simulink model "CoolingPredictiveMaintenance"  (R2024a)
settings: Solver=VariableStepAuto  StartTime=0.0  StopTime=10.0  RelTol=1e-3
settings Model: Creator=deshm  LastModifiedBy=deshm

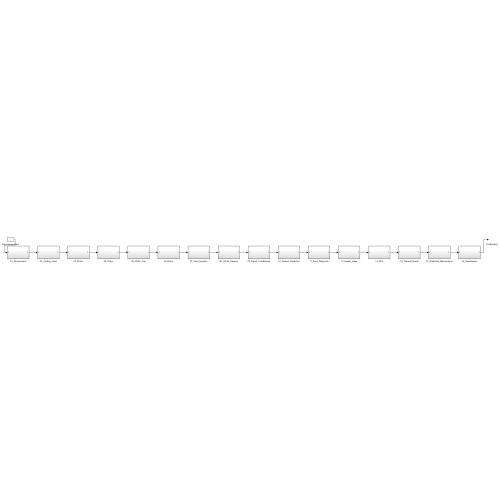
[thumbnail: Simulink's stored preview of the top-level diagram]
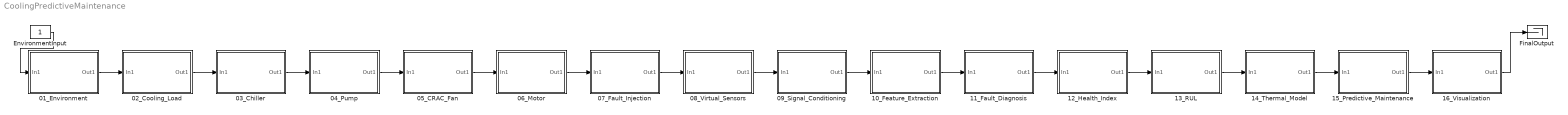
== system CoolingPredictiveMaintenance ==
  01_Environment : Subsystem
  02_Cooling_Load : Subsystem
  03_Chiller : Subsystem
  04_Pump : Subsystem
  05_CRAC_Fan : Subsystem
  06_Motor : Subsystem
  07_Fault_Injection : Subsystem
  08_Virtual_Sensors : Subsystem
  09_Signal_Conditioning : Subsystem
  10_Feature_Extraction : Subsystem
  11_Fault_Diagnosis : Subsystem
  12_Health_Index : Subsystem
  13_RUL : Subsystem
  14_Thermal_Model : Subsystem
  15_Predictive_Maintenance : Subsystem
  16_Visualization : Subsystem
  EnvironmentInput : Constant
  FinalOutput : Terminator
  wires:
  01_Environment/1(Out1) -> 02_Cooling_Load/1(In1)
  02_Cooling_Load/1(Out1) -> 03_Chiller/1(In1)
  03_Chiller/1(Out1) -> 04_Pump/1(In1)
  04_Pump/1(Out1) -> 05_CRAC_Fan/1(In1)
  05_CRAC_Fan/1(Out1) -> 06_Motor/1(In1)
  06_Motor/1(Out1) -> 07_Fault_Injection/1(In1)
  07_Fault_Injection/1(Out1) -> 08_Virtual_Sensors/1(In1)
  08_Virtual_Sensors/1(Out1) -> 09_Signal_Conditioning/1(In1)
  09_Signal_Conditioning/1(Out1) -> 10_Feature_Extraction/1(In1)
  10_Feature_Extraction/1(Out1) -> 11_Fault_Diagnosis/1(In1)
  11_Fault_Diagnosis/1(Out1) -> 12_Health_Index/1(In1)
  12_Health_Index/1(Out1) -> 13_RUL/1(In1)
  13_RUL/1(Out1) -> 14_Thermal_Model/1(In1)
  14_Thermal_Model/1(Out1) -> 15_Predictive_Maintenance/1(In1)
  15_Predictive_Maintenance/1(Out1) -> 16_Visualization/1(In1)
  EnvironmentInput/1 -> 01_Environment/1(In1)
  16_Visualization/1(Out1) -> FinalOutput/1

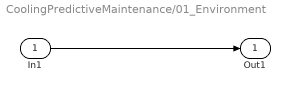
== system CoolingPredictiveMaintenance/01_Environment ==
  In1 : Inport
  Out1 : Outport
  wires:
  In1/1 -> Out1/1

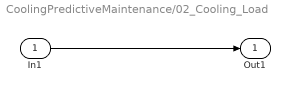
== system CoolingPredictiveMaintenance/02_Cooling_Load ==
  In1 : Inport
  Out1 : Outport
  wires:
  In1/1 -> Out1/1

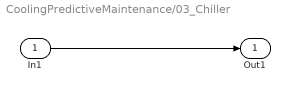
== system CoolingPredictiveMaintenance/03_Chiller ==
  In1 : Inport
  Out1 : Outport
  wires:
  In1/1 -> Out1/1

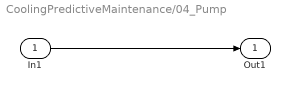
== system CoolingPredictiveMaintenance/04_Pump ==
  In1 : Inport
  Out1 : Outport
  wires:
  In1/1 -> Out1/1

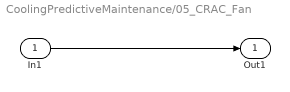
== system CoolingPredictiveMaintenance/05_CRAC_Fan ==
  In1 : Inport
  Out1 : Outport
  wires:
  In1/1 -> Out1/1

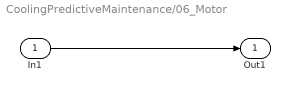
== system CoolingPredictiveMaintenance/06_Motor ==
  In1 : Inport
  Out1 : Outport
  wires:
  In1/1 -> Out1/1

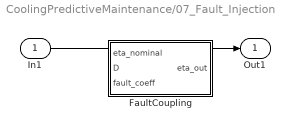
== system CoolingPredictiveMaintenance/07_Fault_Injection ==
  In1 : Inport
  FaultCoupling : MATLAB Function  TreatAsAtomicUnit=on
  Out1 : Outport
  wires:
  In1/1 -> Out1/1

== system CoolingPredictiveMaintenance/08_Virtual_Sensors ==
  In1 : Inport
  Out1 : Outport
  wires:
  In1/1 -> Out1/1

== system CoolingPredictiveMaintenance/09_Signal_Conditioning ==
  In1 : Inport
  Out1 : Outport
  wires:
  In1/1 -> Out1/1

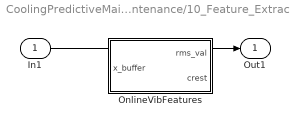
== system CoolingPredictiveMaintenance/10_Feature_Extraction ==
  In1 : Inport
  OnlineVibFeatures : MATLAB Function  TreatAsAtomicUnit=on
  Out1 : Outport
  wires:
  In1/1 -> Out1/1

== system CoolingPredictiveMaintenance/11_Fault_Diagnosis ==
  In1 : Inport
  Out1 : Outport
  wires:
  In1/1 -> Out1/1

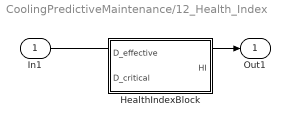
== system CoolingPredictiveMaintenance/12_Health_Index ==
  In1 : Inport
  HealthIndexBlock : MATLAB Function  TreatAsAtomicUnit=on
  Out1 : Outport
  wires:
  In1/1 -> Out1/1

== system CoolingPredictiveMaintenance/13_RUL ==
  In1 : Inport
  Out1 : Outport
  wires:
  In1/1 -> Out1/1

== system CoolingPredictiveMaintenance/14_Thermal_Model ==
  In1 : Inport
  Out1 : Outport
  wires:
  In1/1 -> Out1/1

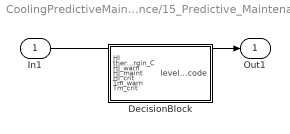
== system CoolingPredictiveMaintenance/15_Predictive_Maintenance ==
  In1 : Inport
  DecisionBlock : MATLAB Function  TreatAsAtomicUnit=on
  Out1 : Outport
  wires:
  In1/1 -> Out1/1

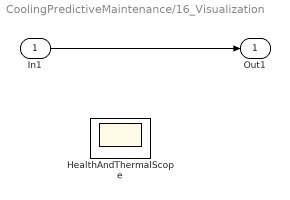
== system CoolingPredictiveMaintenance/16_Visualization ==
  In1 : Inport
  HealthAndThermalScope : Scope
  Out1 : Outport
  wires:
  In1/1 -> Out1/1

== matlab function CoolingPredictiveMaintenance/10_Feature_Extraction/OnlineVibFeatures ==
  data: x_buffer input; rms_val output; crest output
function [rms_val, crest] = OnlineVibFeatures(x_buffer)
%#codegen
% Simulink-native subset of src/features/extract_vibration_features.m
% (time-domain only, for real-time use inside the model).
rms_val = sqrt(mean(x_buffer.^2));
peak = max(abs(x_buffer));
crest = peak / max(rms_val, eps);
end

== matlab function CoolingPredictiveMaintenance/07_Fault_Injection/FaultCoupling ==
  data: eta_nominal input; eta_out output; D input; fault_coeff input
function eta_out = FaultCoupling(eta_nominal, D, fault_coeff)
%#codegen
% Re-expresses the generic degradation coupling from
% src/faults/apply_pump_fault.m / apply_fan_fault.m:
%   eta_fault = eta_nominal * (1 - fault_coeff*D)
eta_out = eta_nominal * (1 - fault_coeff*D);
end

== matlab function CoolingPredictiveMaintenance/12_Health_Index/HealthIndexBlock ==
  data: D_effective input; HI output; D_critical input
function HI = HealthIndexBlock(D_effective, D_critical)
%#codegen
% Re-expresses src/health_index/compute_health_index.m
norm_score = min(max(D_effective / D_critical, 0), 1);
HI = 100 * (1 - norm_score);
end

== matlab function CoolingPredictiveMaintenance/15_Predictive_Maintenance/DecisionBlock ==
  data: HI input; level_code output; thermal_margin_C input; HI_warn input; HI_maint input; HI_crit input; Tm_warn input; Tm_crit input
function level_code = DecisionBlock(HI, thermal_margin_C, HI_warn, HI_maint, HI_crit, Tm_warn, Tm_crit)
%#codegen
% Re-expresses the escalation logic in
% src/maintenance/maintenance_decision_engine.m as a numeric code:
% 0=NORMAL 1=MONITOR 2=WARNING 3=MAINTENANCE_REQUIRED 4=CRITICAL
level_code = 0;
if HI <= HI_crit
    level_code = 4;
elseif HI <= HI_maint
    level_code = max(level_code, 3);
elseif HI <= HI_warn
    level_code = max(level_code, 2);
end
if thermal_margin_C <= Tm_crit
    level_code = 4;
elseif thermal_margin_C <= Tm_warn
    level_code = max(level_code, 2);
end
end
